simulink model "PID_laptop"  (R2026a)
settings: Solver=ode45  StopTime=Tstop  MaxStep=Ts
InitFcn:
  | assert(isscalar(Ts) && isfinite(Ts) && Ts>0, 'Ts must be positive.');
  | assert(isscalar(delay) && isfinite(delay) && delay>=0 && abs(delay/Ts-round(delay/Ts))<1e-9, 'delay must be a nonnegative integer multiple of Ts.');
  | assert(isscalar(u_max) && isfinite(u_max) && u_max>0, 'u_max must be positive.');
  | assert(isequal(size(J),[2 2]) && all(isfinite(J(:))), 'J must be finite 2x2.');
values from neighbouring files (symbols this model uses):
  delay = 0    [init_pid_sim.m]    (also in mws_backup.mat)
  dux = du_base(1)    [init_pid_sim.m]
  duy = du_base(2)    [init_pid_sim.m]
  dx = 0    [init_pid_sim.m]    (also in mws_backup.mat)
  dy = 0    [init_pid_sim.m]    (also in mws_backup.mat)
  Gdx_den = dd    [init_pid_sim.m]
  Gdx_num = nn    [init_pid_sim.m]
  Gdy_den = dd    [init_pid_sim.m]
  Gdy_num = nn    [init_pid_sim.m]
  J = [40.900 -0.296; 0.567 37.800]    [TEST_fine.m]    (also in init_pid_sim.m = [40.900  -0.296; mws_backup.mat = [1  0; 0  1])
  Kd_x = 0    [init_pid_sim.m]    (also in mws_backup.mat)
  Kd_y = 0    [init_pid_sim.m]    (also in mws_backup.mat)
  Ki_x = 20/J(1,1)    [init_pid_sim.m]    (also in mws_backup.mat = 0)
  Ki_y = 20/J(2,2)    [init_pid_sim.m]    (also in mws_backup.mat = 0)
  Kp_x = 0    [init_pid_sim.m]    (also in mws_backup.mat = 0.1)
  Kp_y = 0    [init_pid_sim.m]    (also in mws_backup.mat = 0.1)
  N_x = 100    [init_pid_sim.m]    (also in mws_backup.mat; standard.m = 30; tune_pid.m = 30)
  N_y = 100    [init_pid_sim.m]    (also in mws_backup.mat; standard.m = 30; tune_pid.m = 30)
  step_time = 0.5    [init_pid_sim.m]    (also in mws_backup.mat)
  Ts = cfg.Ts    [PI_opt_estimators_v2.m]    (also in TEST_fine.m = 0.0158; init_pid_sim.m = 0.0158; mws_backup.mat = 0.001)
  u_max = 0.58    [init_pid_sim.m]    (also in mws_backup.mat = 1)
  Xhat_sensor = Xs_sensor    [design_pid.m]    (also in init_pid_sim.m = Xhat_all(est_id, :); standard.m; tune_pid.m)
  Xref = 0    [init_pid_sim.m]    (also in mws_backup.mat)
  Yhat_sensor = Ys_sensor    [design_pid.m]    (also in init_pid_sim.m = Yhat_all(est_id, :); standard.m; tune_pid.m)
  Yref = 0    [init_pid_sim.m]    (also in mws_backup.mat)
undefined symbols (not defined in the file or in its folder): Xs_sensor, Ys_sensor
libraries: slpidlib x2
Description:
  | Standalone MATLAB/Simulink R2026a model. No external M-files required.
  | Edit all parameters in Model Explorer > Model Workspace, then save this SLX.
  | Run button uses these saved values. Logs: SimulationOutput.log_ux/log_uy/log_X/log_Y/log_ex/log_ey.
  | Temporary values only; no hardware identification or gain tuning.
  | Initial unity plant and zero delay create an algebraic loop; tested A-D.
settings Model: Creator=w10  LastModifiedBy=yanmn

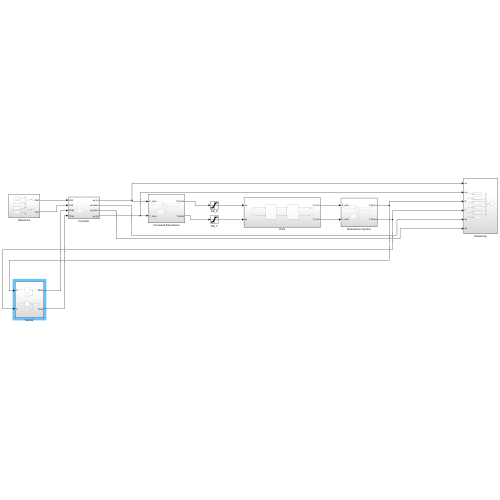
[thumbnail: Simulink's stored preview of the top-level diagram]
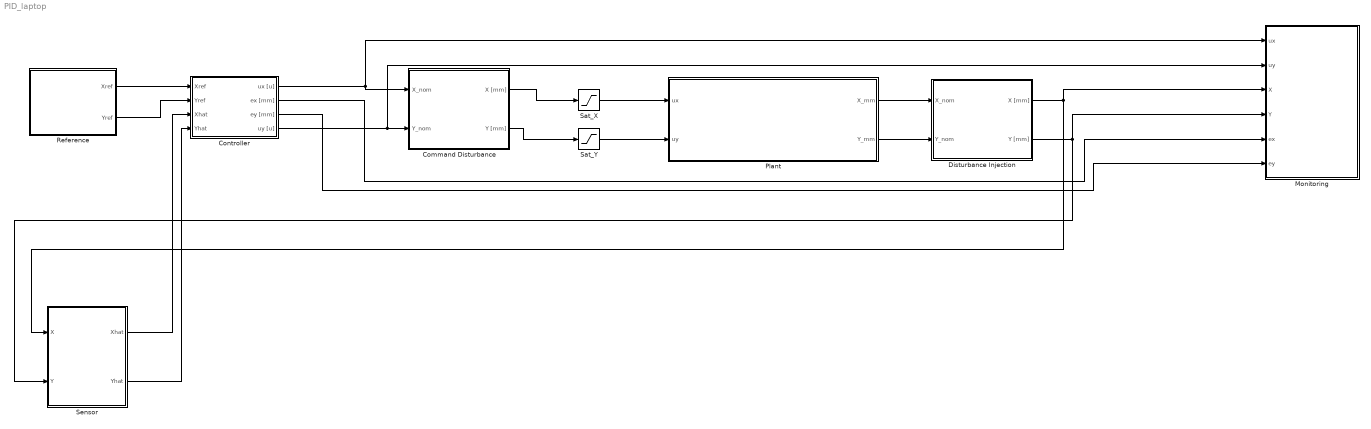
== system PID_laptop ==
  Command Disturbance : Subsystem
  Controller : Subsystem
  Disturbance Injection : Subsystem
  Monitoring : Subsystem
  Plant : Subsystem
  Reference : Subsystem
  Sat_X : Saturate  UpperLimit=u_max  LowerLimit=-u_max
  Sat_Y : Saturate  UpperLimit=u_max  LowerLimit=-u_max
  Sensor : Subsystem
  wires:
  Controller/1(ux [u]) -> Command Disturbance/1(X_nom), Monitoring/1(ux)
  Controller/4(uy [u]) -> Command Disturbance/2(Y_nom), Monitoring/2(uy)
  Reference/1(Xref) -> Controller/1(Xref)
  Reference/2(Yref) -> Controller/2(Yref)
  Sensor/1(Xhat) -> Controller/3(Xhat)
  Sensor/2(Yhat) -> Controller/4(Yhat)
  Controller/2(ex [mm]) -> Monitoring/5(ex)
  Controller/3(ey [mm]) -> Monitoring/6(ey)
  Disturbance Injection/1(X [mm]) -> Monitoring/3(X), Sensor/1(X)
  Disturbance Injection/2(Y [mm]) -> Monitoring/4(Y), Sensor/2(Y)
  Plant/1(X_mm) -> Disturbance Injection/1(X_nom)
  Plant/2(Y_mm) -> Disturbance Injection/2(Y_nom)
  Command Disturbance/1(X [mm]) -> Sat_X/1
  Command Disturbance/2(Y [mm]) -> Sat_Y/1
  Sat_X/1 -> Plant/1(ux)
  Sat_Y/1 -> Plant/2(uy)

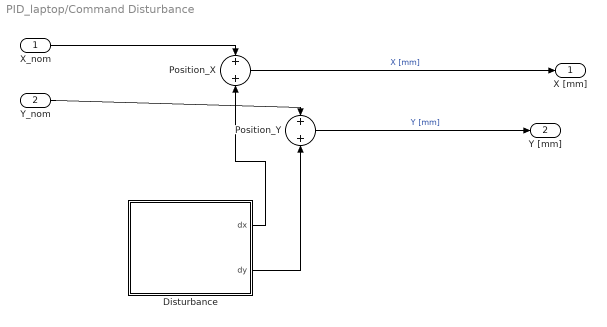
== system PID_laptop/Command Disturbance ==
  X_nom : Inport
  Y_nom : Inport  Port=2
  Disturbance : Subsystem
  Position_X : Sum
  Position_Y : Sum
  X [mm] : Outport
  Y [mm] : Outport  Port=2
  wires:
  Disturbance/2(dy) -> Position_Y/2
  Disturbance/1(dx) -> Position_X/2
  X_nom/1 -> Position_X/1
  Position_X/1 -> X [mm]/1  "X [mm]"
  Position_Y/1 -> Y [mm]/1  "Y [mm]"
  Y_nom/1 -> Position_Y/1

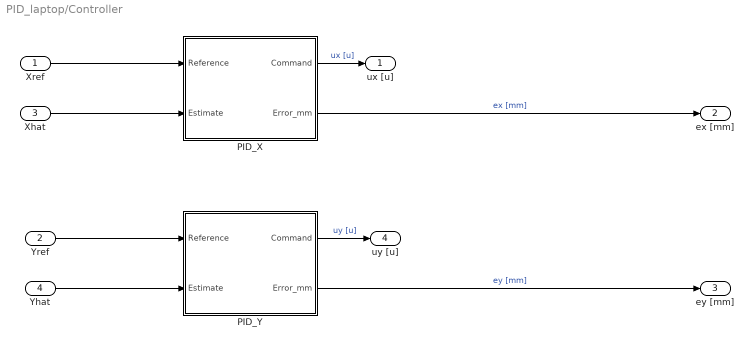
== system PID_laptop/Controller ==
  Xref : Inport
  Yref : Inport  Port=2
  Xhat : Inport  Port=3
  Yhat : Inport  Port=4
  PID_X : Subsystem
  PID_Y : Subsystem
  ux [u] : Outport
  ex [mm] : Outport  Port=2
  ey [mm] : Outport  Port=3
  uy [u] : Outport  Port=4
  wires:
  Xhat/1 -> PID_X/2(Estimate)
  PID_X/2(Error_mm) -> ex [mm]/1  "ex [mm]"
  PID_Y/1(Command) -> uy [u]/1  "uy [u]"
  PID_X/1(Command) -> ux [u]/1  "ux [u]"
  Yhat/1 -> PID_Y/2(Estimate)
  Xref/1 -> PID_X/1(Reference)
  PID_Y/2(Error_mm) -> ey [mm]/1  "ey [mm]"
  Yref/1 -> PID_Y/1(Reference)

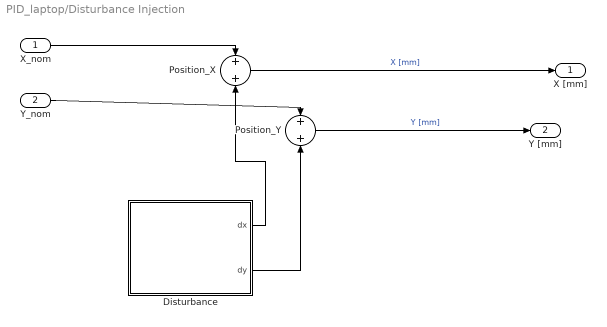
== system PID_laptop/Disturbance Injection ==
  X_nom : Inport
  Y_nom : Inport  Port=2
  Disturbance : Subsystem
  Position_X : Sum
  Position_Y : Sum
  X [mm] : Outport
  Y [mm] : Outport  Port=2
  wires:
  Disturbance/2(dy) -> Position_Y/2
  Disturbance/1(dx) -> Position_X/2
  X_nom/1 -> Position_X/1
  Position_X/1 -> X [mm]/1  "X [mm]"
  Position_Y/1 -> Y [mm]/1  "Y [mm]"
  Y_nom/1 -> Position_Y/1

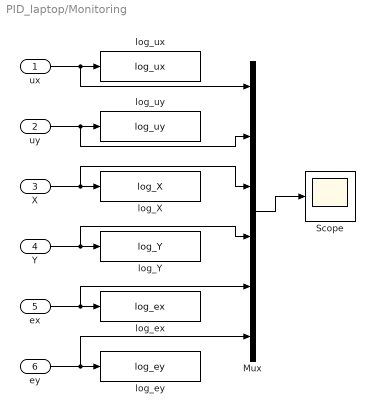
== system PID_laptop/Monitoring ==
  ux : Inport
  uy : Inport  Port=2
  X : Inport  Port=3
  Y : Inport  Port=4
  ex : Inport  Port=5
  ey : Inport  Port=6
  Mux : Mux  Inputs=6
  Scope : Scope
      settings: ActiveDisplayYMinimum=-1  ActiveDisplayYMaximum=1
  log_X : ToWorkspace  VariableName=log_X  SaveFormat=Timeseries  SampleTime=-1
  log_Y : ToWorkspace  VariableName=log_Y  SaveFormat=Timeseries  SampleTime=-1
  log_ex : ToWorkspace  VariableName=log_ex  SaveFormat=Timeseries  SampleTime=-1
  log_ey : ToWorkspace  VariableName=log_ey  SaveFormat=Timeseries  SampleTime=-1
  log_ux : ToWorkspace  VariableName=log_ux  SaveFormat=Timeseries  SampleTime=-1
  log_uy : ToWorkspace  VariableName=log_uy  SaveFormat=Timeseries  SampleTime=-1
  wires:
  Mux/1 -> Scope/1
  ux/1 -> log_ux/1, Mux/1
  uy/1 -> log_uy/1, Mux/2
  X/1 -> log_X/1, Mux/3
  Y/1 -> log_Y/1, Mux/4
  ex/1 -> log_ex/1, Mux/5
  ey/1 -> log_ey/1, Mux/6

== system PID_laptop/Plant ==
  ux : Inport
  uy : Inport  Port=2
  FSM_Dynamics : Subsystem
  Optical_Mapping_J : Subsystem
  X_mm : Outport
  Y_mm : Outport  Port=2
  wires:
  uy/1 -> FSM_Dynamics/2(uy)
  FSM_Dynamics/2(vy) -> Optical_Mapping_J/2(vy)
  ux/1 -> FSM_Dynamics/1(ux)
  Optical_Mapping_J/1(X_mm) -> X_mm/1
  Optical_Mapping_J/2(Y_mm) -> Y_mm/1
  FSM_Dynamics/1(vx) -> Optical_Mapping_J/1(vx)

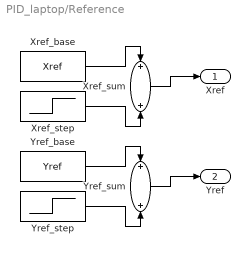
== system PID_laptop/Reference ==
  Xref_base : Constant  Value=Xref
  Xref_step : Step  Time=step_time  FinalValue=Xref_step  SampleTime=Ts
  Xref_sum : Sum
  Yref_base : Constant  Value=Yref
  Yref_step : Step  Time=step_time  FinalValue=Yref_step  SampleTime=Ts
  Yref_sum : Sum
  Xref : Outport
  Yref : Outport  Port=2
  wires:
  Xref_base/1 -> Xref_sum/1
  Xref_step/1 -> Xref_sum/2
  Xref_sum/1 -> Xref/1
  Yref_base/1 -> Yref_sum/1
  Yref_step/1 -> Yref_sum/2
  Yref_sum/1 -> Yref/1

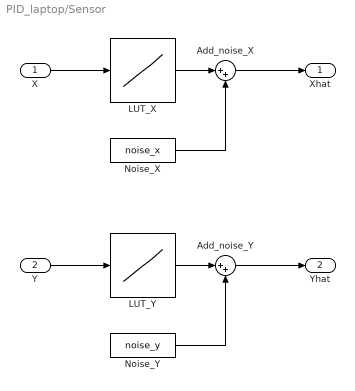
== system PID_laptop/Sensor ==
  X : Inport
  Y : Inport  Port=2
  Add_noise_X : Sum  Inputs=|++
  Add_noise_Y : Sum  Inputs=|++
  LUT_X : Lookup_n-D  NumberOfTableDimensions=1  BreakpointsForDimension1=Xs_sensor  Table=Xhat_sensor  ExtrapMethod=Clip  InternalRulePriority=Speed  RndMeth=Simplest
  LUT_Y : Lookup_n-D  NumberOfTableDimensions=1  BreakpointsForDimension1=Ys_sensor  Table=Yhat_sensor  ExtrapMethod=Clip  InternalRulePriority=Speed  RndMeth=Simplest
  Noise_X : FromWorkspace  VariableName=noise_x  SampleTime=Ts  Interpolate=off  OutputAfterFinalValue=Holding final value
  Noise_Y : FromWorkspace  VariableName=noise_y  SampleTime=Ts  Interpolate=off  OutputAfterFinalValue=Holding final value
  Xhat : Outport
  Yhat : Outport  Port=2
  wires:
  X/1 -> LUT_X/1
  Y/1 -> LUT_Y/1
  LUT_X/1 -> Add_noise_X/1
  Noise_X/1 -> Add_noise_X/2
  Add_noise_X/1 -> Xhat/1
  LUT_Y/1 -> Add_noise_Y/1
  Noise_Y/1 -> Add_noise_Y/2
  Add_noise_Y/1 -> Yhat/1

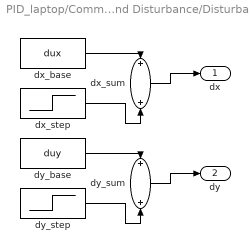
== system PID_laptop/Command Disturbance/Disturbance ==
  dx_base : Constant  Value=dux
  dx_step : Step  Time=step_time  FinalValue=dux_step  SampleTime=Ts
  dx_sum : Sum
  dy_base : Constant  Value=duy
  dy_step : Step  Time=step_time  FinalValue=duy_step  SampleTime=Ts
  dy_sum : Sum
  dx : Outport
  dy : Outport  Port=2
  wires:
  dx_base/1 -> dx_sum/1
  dx_step/1 -> dx_sum/2
  dx_sum/1 -> dx/1
  dy_base/1 -> dy_sum/1
  dy_step/1 -> dy_sum/2
  dy_sum/1 -> dy/1

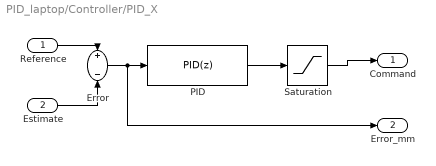
== system PID_laptop/Controller/PID_X ==
  Reference : Inport
  Estimate : Inport  Port=2
  Error : Sum  Inputs=+-
  PID : slpidlib/PID Controller  Controller=PID  Form=Parallel  TimeDomain=Discrete-time  UseExternalTs=off  SampleTime=Ts  IntegratorMethod=Backward Euler  FilterMethod=Backward Euler  ControllerParametersSource=internal  P=Kp_x  I=Ki_x  UseKiTs=off  D=Kd_x  UseExternalDerivativeSource=off  N=N_x  UseFilter=on  TunerSelectOption=Transfer Function Based (PID Tuner App)  InitialConditionSource=internal  InitialConditionForIntegrator=0  InitialConditionForFilter=0  DifferentiatorICPrevScaledInput=0  ExternalReset=none  TrackingMode=off  Kt=1  LimitOutput=on  SatLimitsSource=internal  UpperSaturationLimit=u_max  LowerSaturationLimit=-u_max  LinearizeAsGain=off  AntiWindupMode=clamping  Kb=1  LimitIntegrator=off  UpperIntegratorSaturationLimit=inf  LowerIntegratorSaturationLimit=-inf  POutMin=[]  POutMax=[]  IOutMin=[]  IOutMax=[]  DOutMin=[]  DOutMax=[]  NOutMin=[]  NOutMax=[]  SumOutMin=[]  SumOutMax=[]  SaturationOutMin=[]  SaturationOutMax=[]  PParamMin=[]  PParamMax=[]  IParamMin=[]  IParamMax=[]  DParamMin=[]  DParamMax=[]  NParamMin=[]  NParamMax=[]  KbParamMin=[]  KbParamMax=[]  KtParamMin=[]  KtParamMax=[]  KbOutMin=[]  KbOutMax=[]  KtOutMin=[]  KtOutMax=[]  IntegratorOutMin=[]  IntegratorOutMax=[]  FilterOutMin=[]  FilterOutMax=[]  SumI1OutMin=[]  SumI1OutMax=[]  SumI2OutMin=[]  SumI2OutMax=[]  SumI3OutMin=[]  SumI3OutMax=[]  SumI4OutMin=[]  SumI4OutMax=[]  SumDOutMin=[]  SumDOutMax=[]  DifferentiatorOutMin=[]  DifferentiatorOutMax=[]  FilterDiffOutCoefMin=[]  FilterDiffOutCoefMax=[]  ReciprocalOutMin=[]  ReciprocalOutMax=[]  SumDenOutMin=[]  SumDenOutMax=[]  SumNumOutMin=[]  SumNumOutMax=[]  DivideOutMin=[]  DivideOutMax=[]  UdiffTsProdOutMin=[]  UdiffTsProdOutMax=[]  NTsProdOutMin=[]  NTsProdOutMax=[]  UintegralTsProdOutMin=[]  UintegralTsProdOutMax=[]  UngainTsProdOutMin=[]  UngainTsProdOutMax=[]  ClampingZeroOutDataTypeStr=Inherit: Inherit via back propagation  ClampingZeroOutMin=[]  ClampingZeroOutMax=[]  FilterDenConstantOutDataTypeStr=Inherit: Inherit via back propagation  FilterDenConstantOutMin=[]  FilterDenConstantOutMax=[]  PCopyOutDataTypeStr=Inherit: Inherit via back propagation  PCopyOutMin=[]  PCopyOutMax=[]  NCopyOutDataTypeStr=Inherit: Inherit via back propagation  NCopyOutMin=[]  NCopyOutMax=[]  IntegratorContinuousStateAttributes=''  IntegratorStateMustResolveToSignalObject=off  IntegratorRTWStateStorageClass=Auto  FilterContinuousStateAttributes=''  FilterStateMustResolveToSignalObject=off  FilterRTWStateStorageClass=Auto  ParallelPVariant=InternalParameters  IdealPVariant=Disabled  IVariant=InternalParameters  DVariant=InternalParameters  IntegratorVariant=Discrete  SatVariant=Enabled  AWVariant=DiscClampingParallel  PCopyVariant=Disabled  TRVariant=Disabled  FdbkBlocksVariant=Feedback  IdealPFdbkVariant=Passthrough  SatFdbkVariant=Passthrough  DerivativeFilterVariant=BackwardEulerFilter  NVariant=InternalParameters  NCopyVariant=InternalParameters  FilterICVariant=InternalICsFilter  IntegratorICVariant=InternalICs  ExternalResetVariant=Disabled  TRSumVariant=Passthrough  SumFdbkVariant=Enabled  SumVariant=Sum_PID  TsampFilterVariant=InternalTs  TsampNgainVariant=Passthrough  TsampIntegralVariant=Disabled_SignalSpec  ExternalSaturationOutDataTypeStr=Inherit: Same as second input  DerivativeSourceVariant=ErrorSignal  PreIntVariant=InternalPreInt
      settings: LibrarySourceBlock=simulink/Discrete/Discrete PID Controller
  Saturation : Saturate  UpperLimit=u_max  LowerLimit=-u_max
  Command : Outport
  Error_mm : Outport  Port=2
  wires:
  Reference/1 -> Error/1
  Estimate/1 -> Error/2
  Error/1 -> PID/1, Error_mm/1
  PID/1 -> Saturation/1
  Saturation/1 -> Command/1

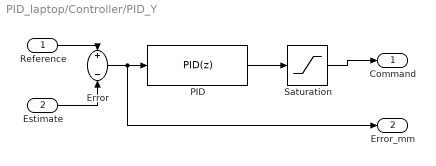
== system PID_laptop/Controller/PID_Y ==
  Reference : Inport
  Estimate : Inport  Port=2
  Error : Sum  Inputs=+-
  PID : slpidlib/PID Controller  Controller=PID  Form=Parallel  TimeDomain=Discrete-time  UseExternalTs=off  SampleTime=Ts  IntegratorMethod=Backward Euler  FilterMethod=Backward Euler  ControllerParametersSource=internal  P=Kp_y  I=Ki_y  UseKiTs=off  D=Kd_y  UseExternalDerivativeSource=off  N=N_y  UseFilter=on  TunerSelectOption=Transfer Function Based (PID Tuner App)  InitialConditionSource=internal  InitialConditionForIntegrator=0  InitialConditionForFilter=0  DifferentiatorICPrevScaledInput=0  ExternalReset=none  TrackingMode=off  Kt=1  LimitOutput=on  SatLimitsSource=internal  UpperSaturationLimit=u_max  LowerSaturationLimit=-u_max  LinearizeAsGain=off  AntiWindupMode=clamping  Kb=1  LimitIntegrator=off  UpperIntegratorSaturationLimit=inf  LowerIntegratorSaturationLimit=-inf  POutMin=[]  POutMax=[]  IOutMin=[]  IOutMax=[]  DOutMin=[]  DOutMax=[]  NOutMin=[]  NOutMax=[]  SumOutMin=[]  SumOutMax=[]  SaturationOutMin=[]  SaturationOutMax=[]  PParamMin=[]  PParamMax=[]  IParamMin=[]  IParamMax=[]  DParamMin=[]  DParamMax=[]  NParamMin=[]  NParamMax=[]  KbParamMin=[]  KbParamMax=[]  KtParamMin=[]  KtParamMax=[]  KbOutMin=[]  KbOutMax=[]  KtOutMin=[]  KtOutMax=[]  IntegratorOutMin=[]  IntegratorOutMax=[]  FilterOutMin=[]  FilterOutMax=[]  SumI1OutMin=[]  SumI1OutMax=[]  SumI2OutMin=[]  SumI2OutMax=[]  SumI3OutMin=[]  SumI3OutMax=[]  SumI4OutMin=[]  SumI4OutMax=[]  SumDOutMin=[]  SumDOutMax=[]  DifferentiatorOutMin=[]  DifferentiatorOutMax=[]  FilterDiffOutCoefMin=[]  FilterDiffOutCoefMax=[]  ReciprocalOutMin=[]  ReciprocalOutMax=[]  SumDenOutMin=[]  SumDenOutMax=[]  SumNumOutMin=[]  SumNumOutMax=[]  DivideOutMin=[]  DivideOutMax=[]  UdiffTsProdOutMin=[]  UdiffTsProdOutMax=[]  NTsProdOutMin=[]  NTsProdOutMax=[]  UintegralTsProdOutMin=[]  UintegralTsProdOutMax=[]  UngainTsProdOutMin=[]  UngainTsProdOutMax=[]  ClampingZeroOutDataTypeStr=Inherit: Inherit via back propagation  ClampingZeroOutMin=[]  ClampingZeroOutMax=[]  FilterDenConstantOutDataTypeStr=Inherit: Inherit via back propagation  FilterDenConstantOutMin=[]  FilterDenConstantOutMax=[]  PCopyOutDataTypeStr=Inherit: Inherit via back propagation  PCopyOutMin=[]  PCopyOutMax=[]  NCopyOutDataTypeStr=Inherit: Inherit via back propagation  NCopyOutMin=[]  NCopyOutMax=[]  IntegratorContinuousStateAttributes=''  IntegratorStateMustResolveToSignalObject=off  IntegratorRTWStateStorageClass=Auto  FilterContinuousStateAttributes=''  FilterStateMustResolveToSignalObject=off  FilterRTWStateStorageClass=Auto  ParallelPVariant=InternalParameters  IdealPVariant=Disabled  IVariant=InternalParameters  DVariant=InternalParameters  IntegratorVariant=Discrete  SatVariant=Enabled  AWVariant=DiscClampingParallel  PCopyVariant=Disabled  TRVariant=Disabled  FdbkBlocksVariant=Feedback  IdealPFdbkVariant=Passthrough  SatFdbkVariant=Passthrough  DerivativeFilterVariant=BackwardEulerFilter  NVariant=InternalParameters  NCopyVariant=InternalParameters  FilterICVariant=InternalICsFilter  IntegratorICVariant=InternalICs  ExternalResetVariant=Disabled  TRSumVariant=Passthrough  SumFdbkVariant=Enabled  SumVariant=Sum_PID  TsampFilterVariant=InternalTs  TsampNgainVariant=Passthrough  TsampIntegralVariant=Disabled_SignalSpec  ExternalSaturationOutDataTypeStr=Inherit: Same as second input  DerivativeSourceVariant=ErrorSignal  PreIntVariant=InternalPreInt
      settings: LibrarySourceBlock=simulink/Discrete/Discrete PID Controller
  Saturation : Saturate  UpperLimit=u_max  LowerLimit=-u_max
  Command : Outport
  Error_mm : Outport  Port=2
  wires:
  Reference/1 -> Error/1
  Estimate/1 -> Error/2
  Error/1 -> PID/1, Error_mm/1
  PID/1 -> Saturation/1
  Saturation/1 -> Command/1

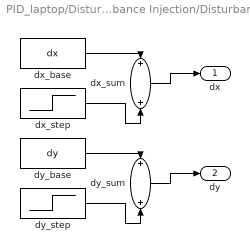
== system PID_laptop/Disturbance Injection/Disturbance ==
  dx_base : Constant  Value=dx
  dx_step : Step  Time=step_time  FinalValue=dx_step  SampleTime=Ts
  dx_sum : Sum
  dy_base : Constant  Value=dy
  dy_step : Step  Time=step_time  FinalValue=dy_step  SampleTime=Ts
  dy_sum : Sum
  dx : Outport
  dy : Outport  Port=2
  wires:
  dx_base/1 -> dx_sum/1
  dx_step/1 -> dx_sum/2
  dx_sum/1 -> dx/1
  dy_base/1 -> dy_sum/1
  dy_step/1 -> dy_sum/2
  dy_sum/1 -> dy/1

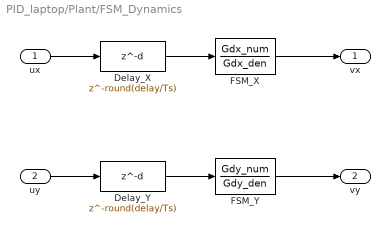
== system PID_laptop/Plant/FSM_Dynamics ==
  ux : Inport
  uy : Inport  Port=2
  Delay_X : Delay  DelayLength=round(delay/Ts)  SampleTime=Ts
  Delay_Y : Delay  DelayLength=round(delay/Ts)  SampleTime=Ts
  FSM_X : DiscreteTransferFcn  Numerator=Gdx_num  Denominator=Gdx_den
  FSM_Y : DiscreteTransferFcn  Numerator=Gdy_num  Denominator=Gdy_den
  vx : Outport
  vy : Outport  Port=2
  wires:
  ux/1 -> Delay_X/1
  Delay_X/1 -> FSM_X/1
  FSM_X/1 -> vx/1
  uy/1 -> Delay_Y/1
  Delay_Y/1 -> FSM_Y/1
  FSM_Y/1 -> vy/1

== system PID_laptop/Plant/Optical_Mapping_J ==
  vx : Inport
  vy : Inport  Port=2
  Demux : Demux  Outputs=2
  J : Gain  Gain=J  Multiplication=Matrix(K*u)
  Mux : Mux  Inputs=2
  X_mm : Outport
  Y_mm : Outport  Port=2
  wires:
  vx/1 -> Mux/1
  vy/1 -> Mux/2
  Mux/1 -> J/1
  J/1 -> Demux/1
  Demux/1 -> X_mm/1
  Demux/2 -> Y_mm/1
